simulink model "PartC"  (R2022b)
settings: Solver=ode4  StartTime=0.0  StopTime=1  FixedStep=0.001  RelTol=1e-3
libraries: slpidlib x2
settings Model: PacingRate=0.100000  Creator=Dimuthu  LastModifiedBy=Mushrif
settings DebuggingCC: UnconnectedInputMsg=warning  UnconnectedOutputMsg=warning  UnconnectedLineMsg=warning
settings ModelReferenceCC: EnableRefExpFcnMdlSchedulingChecks=on
settings RTWCC: DLArmComputeVersion=19.05

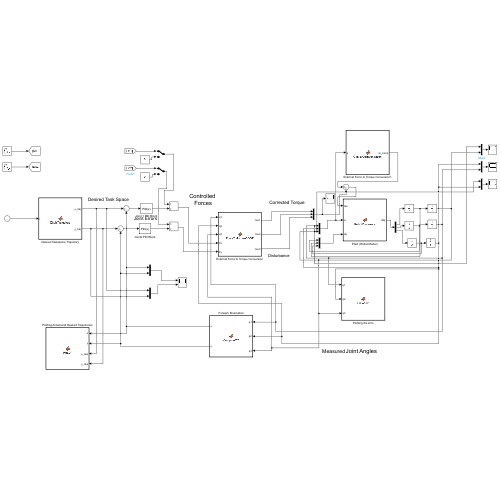
[thumbnail: Simulink's stored preview of the top-level diagram]
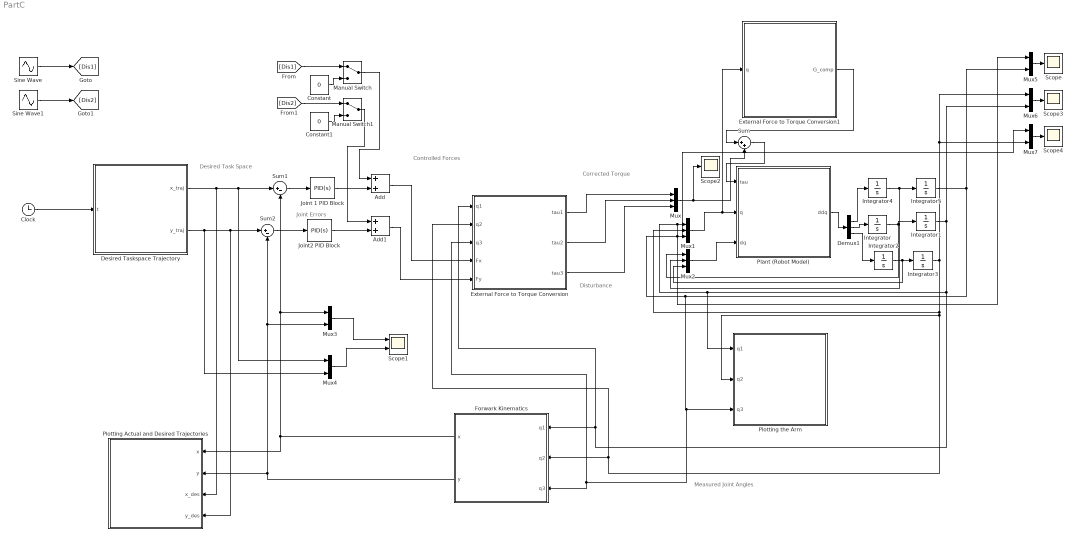
== system PartC ==
  note: Corrected Torque
  note: Disturbance
  note: Measured Joint Angles
  note: Desired Task Space
  note: Controlled
      | Forces
  note: Joint Errors
  Add : Sum
  Add1 : Sum
  Clock : Clock
  Constant : Constant  Value=0
  Constant1 : Constant  Value=0
  Demux1 : Demux  Outputs=3
  Desired Taskspace Trajectory : MATLAB Function  TreatAsAtomicUnit=on
  External Force to Torque Conversion : MATLAB Function  TreatAsAtomicUnit=on
  External Force to Torque Conversion1 : MATLAB Function  TreatAsAtomicUnit=on
  Forwark Kinematics : MATLAB Function  TreatAsAtomicUnit=on
  Integrator{,1..5} (6 alike) : Integrator
  Joint 1 PID Block : slpidlib/PID Controller  Controller=PID  Form=Parallel  TimeDomain=Continuous-time  UseExternalTs=off  SampleTime=-1  IntegratorMethod=Forward Euler  FilterMethod=Forward Euler  ControllerParametersSource=internal  P=100  I=0  UseKiTs=off  D=0  N=100  UseFilter=on  TunerSelectOption=Transfer Function Based (PID Tuner App)  InitialConditionSource=internal  InitialConditionForIntegrator=0  InitialConditionForFilter=0  DifferentiatorICPrevScaledInput=0  ExternalReset=none  TrackingMode=off  Kt=1  LimitOutput=off  SatLimitsSource=internal  UpperSaturationLimit=inf  LowerSaturationLimit=-inf  LinearizeAsGain=on  AntiWindupMode=none  Kb=1  LimitIntegrator=off  UpperIntegratorSaturationLimit=inf  LowerIntegratorSaturationLimit=-inf  POutMin=[]  POutMax=[]  IOutMin=[]  IOutMax=[]  DOutMin=[]  DOutMax=[]  NOutMin=[]  NOutMax=[]  SumOutMin=[]  SumOutMax=[]  SaturationOutMin=[]  SaturationOutMax=[]  PParamMin=[]  PParamMax=[]  IParamMin=[]  IParamMax=[]  DParamMin=[]  DParamMax=[]  NParamMin=[]  NParamMax=[]  KbParamMin=[]  KbParamMax=[]  KtParamMin=[]  KtParamMax=[]  KbOutMin=[]  KbOutMax=[]  KtOutMin=[]  KtOutMax=[]  IntegratorOutMin=[]  IntegratorOutMax=[]  FilterOutMin=[]  FilterOutMax=[]  SumI1OutMin=[]  SumI1OutMax=[]  SumI2OutMin=[]  SumI2OutMax=[]  SumI3OutMin=[]  SumI3OutMax=[]  SumI4OutMin=[]  SumI4OutMax=[]  SumDOutMin=[]  SumDOutMax=[]  DifferentiatorOutMin=[]  DifferentiatorOutMax=[]  FilterDiffOutCoefMin=[]  FilterDiffOutCoefMax=[]  ReciprocalOutMin=[]  ReciprocalOutMax=[]  SumDenOutMin=[]  SumDenOutMax=[]  SumNumOutMin=[]  SumNumOutMax=[]  DivideOutMin=[]  DivideOutMax=[]  UdiffTsProdOutMin=[]  UdiffTsProdOutMax=[]  NTsProdOutMin=[]  NTsProdOutMax=[]  UintegralTsProdOutMin=[]  UintegralTsProdOutMax=[]  UngainTsProdOutMin=[]  UngainTsProdOutMax=[]  ClampingZeroOutDataTypeStr=Inherit: Inherit via back propagation  ClampingZeroOutMin=[]  ClampingZeroOutMax=[]  FilterDenConstantOutDataTypeStr=Inherit: Inherit via back propagation  FilterDenConstantOutMin=[]  FilterDenConstantOutMax=[]  PCopyOutDataTypeStr=Inherit: Inherit via back propagation  PCopyOutMin=[]  PCopyOutMax=[]  NCopyOutDataTypeStr=Inherit: Inherit via back propagation  NCopyOutMin=[]  NCopyOutMax=[]  IntegratorContinuousStateAttributes=''  IntegratorStateMustResolveToSignalObject=off  IntegratorRTWStateStorageClass=Auto  FilterContinuousStateAttributes=''  FilterStateMustResolveToSignalObject=off  FilterRTWStateStorageClass=Auto  ParallelPVariant=InternalParameters  IdealPVariant=Disabled  IVariant=InternalParameters  DVariant=InternalParameters  IntegratorVariant=Continuous  SatVariant=Disabled  AWVariant=Passthrough  PCopyVariant=Disabled  TRVariant=Disabled  FdbkBlocksVariant=Forward  IdealPFdbkVariant=Disabled  SatFdbkVariant=Disabled  DerivativeFilterVariant=ContFilter  NVariant=InternalParameters  NCopyVariant=Disabled  FilterICVariant=InternalICsFilter  IntegratorICVariant=InternalICs  ExternalResetVariant=Disabled  TRSumVariant=Passthrough  SumFdbkVariant=Disabled  SumVariant=Sum_PID  TsampFilterVariant=InternalTs  TsampNgainVariant=Passthrough  TsampIntegralVariant=Passthrough  ExternalSaturationOutDataTypeStr=Inherit: Same as second input
  Joint2 PID Block : slpidlib/PID Controller  Controller=PID  Form=Parallel  TimeDomain=Continuous-time  UseExternalTs=off  SampleTime=-1  IntegratorMethod=Forward Euler  FilterMethod=Forward Euler  ControllerParametersSource=internal  P=10  I=0  UseKiTs=off  D=0  N=100  UseFilter=on  TunerSelectOption=Transfer Function Based (PID Tuner App)  InitialConditionSource=internal  InitialConditionForIntegrator=0  InitialConditionForFilter=0  DifferentiatorICPrevScaledInput=0  ExternalReset=none  TrackingMode=off  Kt=1  LimitOutput=off  SatLimitsSource=internal  UpperSaturationLimit=inf  LowerSaturationLimit=-inf  LinearizeAsGain=on  AntiWindupMode=none  Kb=1  LimitIntegrator=off  UpperIntegratorSaturationLimit=inf  LowerIntegratorSaturationLimit=-inf  POutMin=[]  POutMax=[]  IOutMin=[]  IOutMax=[]  DOutMin=[]  DOutMax=[]  NOutMin=[]  NOutMax=[]  SumOutMin=[]  SumOutMax=[]  SaturationOutMin=[]  SaturationOutMax=[]  PParamMin=[]  PParamMax=[]  IParamMin=[]  IParamMax=[]  DParamMin=[]  DParamMax=[]  NParamMin=[]  NParamMax=[]  KbParamMin=[]  KbParamMax=[]  KtParamMin=[]  KtParamMax=[]  KbOutMin=[]  KbOutMax=[]  KtOutMin=[]  KtOutMax=[]  IntegratorOutMin=[]  IntegratorOutMax=[]  FilterOutMin=[]  FilterOutMax=[]  SumI1OutMin=[]  SumI1OutMax=[]  SumI2OutMin=[]  SumI2OutMax=[]  SumI3OutMin=[]  SumI3OutMax=[]  SumI4OutMin=[]  SumI4OutMax=[]  SumDOutMin=[]  SumDOutMax=[]  DifferentiatorOutMin=[]  DifferentiatorOutMax=[]  FilterDiffOutCoefMin=[]  FilterDiffOutCoefMax=[]  ReciprocalOutMin=[]  ReciprocalOutMax=[]  SumDenOutMin=[]  SumDenOutMax=[]  SumNumOutMin=[]  SumNumOutMax=[]  DivideOutMin=[]  DivideOutMax=[]  UdiffTsProdOutMin=[]  UdiffTsProdOutMax=[]  NTsProdOutMin=[]  NTsProdOutMax=[]  UintegralTsProdOutMin=[]  UintegralTsProdOutMax=[]  UngainTsProdOutMin=[]  UngainTsProdOutMax=[]  ClampingZeroOutDataTypeStr=Inherit: Inherit via back propagation  ClampingZeroOutMin=[]  ClampingZeroOutMax=[]  FilterDenConstantOutDataTypeStr=Inherit: Inherit via back propagation  FilterDenConstantOutMin=[]  FilterDenConstantOutMax=[]  PCopyOutDataTypeStr=Inherit: Inherit via back propagation  PCopyOutMin=[]  PCopyOutMax=[]  NCopyOutDataTypeStr=Inherit: Inherit via back propagation  NCopyOutMin=[]  NCopyOutMax=[]  IntegratorContinuousStateAttributes=''  IntegratorStateMustResolveToSignalObject=off  IntegratorRTWStateStorageClass=Auto  FilterContinuousStateAttributes=''  FilterStateMustResolveToSignalObject=off  FilterRTWStateStorageClass=Auto  ParallelPVariant=InternalParameters  IdealPVariant=Disabled  IVariant=InternalParameters  DVariant=InternalParameters  IntegratorVariant=Continuous  SatVariant=Disabled  AWVariant=Passthrough  PCopyVariant=Disabled  TRVariant=Disabled  FdbkBlocksVariant=Forward  IdealPFdbkVariant=Disabled  SatFdbkVariant=Disabled  DerivativeFilterVariant=ContFilter  NVariant=InternalParameters  NCopyVariant=Disabled  FilterICVariant=InternalICsFilter  IntegratorICVariant=InternalICs  ExternalResetVariant=Disabled  TRSumVariant=Passthrough  SumFdbkVariant=Disabled  SumVariant=Sum_PID  TsampFilterVariant=InternalTs  TsampNgainVariant=Passthrough  TsampIntegralVariant=Passthrough  ExternalSaturationOutDataTypeStr=Inherit: Same as second input
  Manual Switch : ManualSwitch
  Manual Switch1 : ManualSwitch
  Mux : Mux  Inputs=3
  Mux1 : Mux  Inputs=3
  Mux2 : Mux  Inputs=3
  Mux{3..7} (5 alike) : Mux  Inputs=2
  Plant (Robot Model) : MATLAB Function  TreatAsAtomicUnit=on
  Plotting Actual and Desired Trajectories : MATLAB Function  TreatAsAtomicUnit=on
  Plotting the Arm : MATLAB Function  TreatAsAtomicUnit=on
  Scope{,2..4} (4 alike) : Scope
  Scope1 : Scope  NumInputPorts=2
  Sine Wave : Sin  Amplitude=0.1  SampleTime=0
  Sine Wave1 : Sin  Amplitude=0.05  SampleTime=0
  Sum : Sum  Inputs=|++
  Sum1 : Sum  Inputs=|+-
  Sum2 : Sum  Inputs=|+-
  wires:
  Desired Taskspace Trajectory/1(x_traj) -> Plotting Actual and Desired Trajectories/3(x_des), Mux4/1, Sum1/1
  Desired Taskspace Trajectory/2(y_traj) -> Mux4/2, Plotting Actual and Desired Trajectories/4(y_des), Sum2/1
  Forwark Kinematics/1(x) -> Mux3/1, Sum1/2, Plotting Actual and Desired Trajectories/1(x)
  Forwark Kinematics/2(y) -> Plotting Actual and Desired Trajectories/2(y), Mux3/2, Sum2/2
  Sum2/1 -> Joint2 PID Block/1
  Sum1/1 -> Joint 1 PID Block/1
  External Force to Torque Conversion/1(tau1) -> Mux/1
  Integrator/1 -> Integrator1/1, Mux2/1
  Demux1/2 -> Integrator/1
  Demux1/3 -> Integrator2/1
  Integrator2/1 -> Mux2/3, Integrator3/1
  Mux1/1 -> External Force to Torque Conversion1/1(q), Plant (Robot Model)/2(q)
  Mux2/1 -> Plant (Robot Model)/3(dq)
  Integrator1/1 -> Mux6/2, Mux5/1, Mux1/1, Plotting the Arm/1(q1), External Force to Torque Conversion/1(q1), Forwark Kinematics/1(q1)
  Integrator3/1 -> Mux6/1, Mux7/2, Mux1/2, Plotting the Arm/2(q2), External Force to Torque Conversion/2(q2), Forwark Kinematics/2(q2)
  Plant (Robot Model)/1(ddq) -> Demux1/1
  Mux3/1 -> Scope1/1
  Mux4/1 -> Scope1/2
  Mux/1 -> Sum/2, Scope2/1
  External Force to Torque Conversion/2(tau2) -> Mux/2
  Demux1/1 -> Integrator4/1
  Integrator4/1 -> Mux2/2, Integrator5/1
  Integrator5/1 -> Mux5/2, Forwark Kinematics/3(q3), External Force to Torque Conversion/3(q3), Plotting the Arm/3(q3), Mux7/1, Mux1/3
  External Force to Torque Conversion/3(tau3) -> Mux/3
  Clock/1 -> Desired Taskspace Trajectory/1(t)
  External Force to Torque Conversion1/1(G_comp) -> Sum/1
  Sum/1 -> Plant (Robot Model)/1(tau)
  Mux5/1 -> Scope/1
  Mux6/1 -> Scope3/1
  Mux7/1 -> Scope4/1
  Joint2 PID Block/1 -> Add1/2
  Joint 1 PID Block/1 -> Add/2
  Add/1 -> External Force to Torque Conversion/4(Fx)
  Add1/1 -> External Force to Torque Conversion/5(Fy)
  Sine Wave/1 -> [Dis1]
  Sine Wave1/1 -> [Dis2]
  Manual Switch1/1 -> Add1/1
  Manual Switch/1 -> Add/1
  [Dis1] -> Manual Switch/1
  [Dis2] -> Manual Switch1/1
  Constant1/1 -> Manual Switch1/2
  Constant/1 -> Manual Switch/2

== matlab function PartC/Forwark Kinematics ==
  settings: updateMethod=DISCRETE
  data: q1 input double size=1; q2 input double size=1; x output; y output; q3 input
function [x, y] = ComputeXY(q1, q2, q3)
%#codegen

% Define link lengths (can be parameters later)
l1 = 0.5; l2 = 0.4; l3 = 0.3;

% Compute forward kinematics
x = l1 * cos(q1) + l2 * cos(q1 + q2)+ l3 * cos(q1 + q2 + q3);
y = l1 * sin(q1) + l2 * sin(q1 + q2)+ l3 * sin(q1 + q2 + q3);
end

== matlab function PartC/Desired Taskspace Trajectory ==
  settings: updateMethod=DISCRETE
  data: x_traj output; y_traj output; t input
function [x_traj, y_traj] = CircleTrajectory(t)
T = 1;             % total time
%dt = 0.05;          % time step
%t = 0:dt:T;
%N = length(t);

% Robot planar workspace: max reach = 0.5 + 0.4 + 0.3 = 1.2 m
% Set a reachable elliptical trajectory in the XY plane
cx = 0.9; cy = 0.3;           % center of ellipse
rx = 0.3; ry = 0.2;           % radii (x and y)
%rx = 0.8; ry = 0.4; 

% 2D elliptical arc in XY plane
x_traj = cx + rx * cos(2*pi*t/T);
y_traj = cy + ry * sin(2*pi*t/T);
end

== matlab function PartC/External Force to Torque Conversion ==
  settings: updateMethod=DISCRETE
  data: q1 input double size=[1,1]; q2 input double size=[1,1]; q3 input size=[1,1]; tau1 output size=[1,1]; tau2 output size=[1,1]; Fx input size=[1,1]; Fy input size=[1,1]; tau3 output size=[1,1]
function [tau1, tau2, tau3] = ForceToTorque3DOF(q1, q2, q3, Fx, Fy)
% Converts end-effector force to joint torques for a 3-DOF planar robot.
% Safer version without damping or dq input.

% Link lengths
l1 = 0.5; l2 = 0.4; l3 = 0.3;

% === Wrap angles to avoid large angle buildup ===
q1 = wrapToPi(q1);
q2 = wrapToPi(q2);
q3 = wrapToPi(q3);

% === Force saturation to avoid instability ===
Fmax = 100;  % Tune as needed
Fx = max(min(Fx, Fmax), -Fmax);
Fy = max(min(Fy, Fmax), -Fmax);

F_ee = [Fx; Fy];  % Cartesian force

% === Trigonometric precomputations ===
s1 = sin(q1); c1 = cos(q1);
s12 = sin(q1 + q2); c12 = cos(q1 + q2);
s123 = sin(q1 + q2 + q3); c123 = cos(q1 + q2 + q3);

% === Jacobian (2x3) ===
J11 = -l1*s1 - l2*s12 - l3*s123;
J12 =       -l2*s12 - l3*s123;
J13 =                 -l3*s123;

J21 =  l1*c1 + l2*c12 + l3*c123;
J22 =         l2*c12 + l3*c123;
J23 =                  l3*c123;

J = [J11 J12 J13;
     J21 J22 J23];

% === Check Jacobian and force validity ===
if any(~isfinite(J(:))) || any(~isfinite(F_ee))
    tau_vec = [0; 0; 0];  % Failsafe zero torque
else
    tau_vec = J' * F_ee;
end

% === Output joint torques ===
tau1 = tau_vec(1);
tau2 = tau_vec(2);
tau3 = tau_vec(3);
end

== matlab function PartC/Plant (Robot Model) ==
  data: tau input double size=[3,1]; q input double size=[3,1]; dq input size=[3,1]; ddq output size=[3,1]
function ddq = RobotDynamics(tau, q, dq)
% 3-DOF Planar Robot Dynamics - ROBUST VERSION
% Inputs:
%   tau - joint torques [3x1]
%   q   - joint positions [3x1]
%   dq  - joint velocities [3x1]
% Output:
%   ddq - joint accelerations [3x1]

% --- Ensure inputs are column vectors ---
q = q(:);
dq = dq(:);
tau = tau(:);

% --- Robot parameters (MUST MATCH ALL OTHER BLOCKS) ---
m1 = 1; m2 = 1; m3 = 1;
l1 = 0.5; l2 = 0.4; l3 = 0.3;
%l1 = 0.1; l2 = 0.1;l3 = 0.1;
g = 9.81;

% === Inertia Matrix M(q) ===
M11 = m1*l1^2 + m2*(l1^2 + l2^2 + 2*l1*l2*cos(q(2))) + ...
      m3*(l1^2 + l2^2 + l3^2 + 2*l1*l2*cos(q(2)) + 2*l1*l3*cos(q(2)+q(3)) + 2*l2*l3*cos(q(3)));
M12 = m2*(l2^2 + l1*l2*cos(q(2))) + ...
      m3*(l2^2 + l3^2 + l1*l2*cos(q(2)) + l1*l3*cos(q(2)+q(3)) + l2*l3*cos(q(3)));
M13 = m3*(l3^2 + l1*l3*cos(q(2)+q(3)) + l2*l3*cos(q(3)));
M22 = m2*l2^2 + m3*(l2^2 + l3^2 + 2*l2*l3*cos(q(3)));
M23 = m3*(l3^2 + l2*l3*cos(q(3)));
M33 = m3*l3^2;
M = [M11 M12 M13;
     M12 M22 M23;
     M13 M23 M33];

% === Coriolis and Centripetal Matrix C(q,dq) ===
c1 = -m2*l1*l2*sin(q(2))*(2*dq(1)*dq(2) + dq(2)^2) ...
     - m3*(l1*l2*sin(q(2))*(2*dq(1)*dq(2) + dq(2)^2) ...
     + l1*l3*sin(q(2)+q(3))*(2*dq(1)*(dq(2)+dq(3)) + (dq(2)+dq(3))^2) ...
     + l2*l3*sin(q(3))*(2*dq(2)*dq(3) + dq(3)^2));
c2 = m2*l1*l2*sin(q(2))*dq(1)^2 + ...
     m3*(l1*l2*sin(q(2))*dq(1)^2 + ...
     l1*l3*sin(q(2)+q(3))*dq(1)^2 + ...
     l2*l3*sin(q(3))*(2*dq(2)*dq(3) + dq(3)^2));
c3 = m3*(l1*l3*sin(q(2)+q(3))*dq(1)^2 + ...
         l2*l3*sin(q(3))*dq(2)^2);
C = [c1; c2; c3];

% === Gravity Vector G(q) ===
G1 = g*(m1*l1*cos(q(1)) + m2*(l1*cos(q(1)) + l2*cos(q(1)+q(2))) + ...
        m3*(l1*cos(q(1)) + l2*cos(q(1)+q(2)) + l3*cos(q(1)+q(2)+q(3))));
G2 = g*(m2*l2*cos(q(1)+q(2)) + m3*(l2*cos(q(1)+q(2)) + l3*cos(q(1)+q(2)+q(3))));
G3 = g*(m3*l3*cos(q(1)+q(2)+q(3)));
G = [G1; G2; G3];

% =================================================================
% === MODIFICATIONS FOR STABILITY =================================
% =================================================================

% --- MODIFICATION 1: Add Joint Damping ---
% This adds physical realism (friction) and helps stabilize the system.
% Tune these values if needed. Higher values = more "syrupy" motion.
D = diag([0.5, 0.5, 0.5]);
DampingTorque = D * dq;

% --- MODIFICATION 2: Regularize the Inertia Matrix ---
% This is the direct fix for the singularity crash.
% It adds a tiny value to the diagonal of M, guaranteeing it is
% always invertible and preventing the ddq calculation from failing.
epsilon = 1e-6; % A small number
M_reg = M + epsilon * eye(size(M));

% --- Calculate the net torque on the system ---
% We subtract Coriolis, Gravity, and the new Damping torques.
residual_torque = tau - C - G - DampingTorque;

% --- Final Robust Calculation of ddq ---
% Use the regularized matrix M_reg to avoid crashes.
ddq = M_reg \ residual_torque;

% --- Failsafe Guard ---
% If for any reason ddq is still not finite, output zeros to
% prevent the entire simulation from stopping.
if any(~isfinite(ddq))
    ddq = zeros(3,1);
end

end

== matlab function PartC/Plotting the Arm ==
  settings: updateMethod=DISCRETE
  data: q1 input double size=1; q2 input double size=1; q3 input
function DrawArm(q1, q2, q3)
% DrawArm - Plots a 3-DOF planar robot arm in 2D
% Inputs: q1, q2, q3 - joint angles (in radians)

% Link lengths
l1 = 0.5; l2 = 0.4; l3 = 0.3;

% Forward kinematics
x1 = l1 * cos(q1);
y1 = l1 * sin(q1);

x2 = x1 + l2 * cos(q1 + q2);
y2 = y1 + l2 * sin(q1 + q2);

x3 = x2 + l3 * cos(q1 + q2 + q3);
y3 = y2 + l3 * sin(q1 + q2 + q3);

% Persistent graphics handles
persistent h1 h2 h3 base initialized
if isempty(initialized)
    figure(1); clf;
    axis equal; axis([-3.5 3.5 -3.5 3.5]);
    grid on; hold on;
    base = plot(0, 0, 'ko', 'MarkerSize', 6, 'MarkerFaceColor', 'k');
    h1 = plot([0, x1], [0, y1], 'r-', 'LineWidth', 5);       % Link 1
    h2 = plot([x1, x2], [y1, y2], 'g-', 'LineWidth', 5);     % Link 2
    h3 = plot([x2, x3], [y2, y3], 'b-', 'LineWidth', 5);     % Link 3
    initialized = true;
else
    set(h1, 'XData', [0, x1], 'YData', [0, y1]);
    set(h2, 'XData', [x1, x2], 'YData', [y1, y2]);
    set(h3, 'XData', [x2, x3], 'YData', [y2, y3]);
end

drawnow;
end

== matlab function PartC/Plotting Actual and Desired Trajectories ==
  settings: updateMethod=DISCRETE
  data: x input double size=1; y input double size=1; x_des input; y_des input
function PlotXY(x, y, x_des, y_des)
%#codegen

persistent h_actual h_des trail_x trail_y trail_xd trail_yd idx initialized
if isempty(initialized)
    figure(2); clf;
    axis equal; axis([0 2 -1.2 1.2]);
    grid on; hold on;

    h_actual = plot(nan, nan, 'b-', 'LineWidth', 2); % Actual path
    h_des    = plot(nan, nan, 'r--', 'LineWidth', 2); % Desired path

    N = 10000;
    trail_x = nan(N,1);
    trail_y = nan(N,1);
    trail_xd = nan(N,1);
    trail_yd = nan(N,1);
    idx = 1;

    initialized = true;
end

if idx <= length(trail_x)
    trail_x(idx)  = x;
    trail_y(idx)  = y;
    trail_xd(idx) = x_des;
    trail_yd(idx) = y_des;

    set(h_actual, 'XData', trail_x,  'YData', trail_y);
    set(h_des,    'XData', trail_xd, 'YData', trail_yd);

    idx = idx + 1;
end

drawnow limitrate;
end

== matlab function PartC/External Force to Torque Conversion1 ==
  settings: updateMethod=DISCRETE
  data: q input double size=[1,3]; G_comp output size=[3]
function G_comp = GravityCompensation(q)
% Calculates the gravity compensation torque vector G(q).
% This block computes the torques required to hold the robot's
% position against gravity.
%
% Input:
%   q      - A 3x1 vector of current joint angles [q1; q2; q3].
% Output:
%   G_comp - A 3x1 vector of gravity torques [G1; G2; G3].

% --- Ensure input is a column vector to prevent dimension errors ---
% This is a safety measure for Simulink.
q = q(:);

% --- Robot Parameters ---
% IMPORTANT: These parameters MUST exactly match the ones in your
% RobotDynamics.m file for the compensation to be effective.
m1 = 1; m2 = 1; m3 = 1;
l1 = 0.5; l2 = 0.4; l3 = 0.3;
g = 9.81;

% --- Gravity Vector G(q) Calculation ---
% This is the exact same logic as in your RobotDynamics file.
% It calculates the torque on each joint due to gravity.
G1 = g * (m1*l1*cos(q(1)) + m2*(l1*cos(q(1)) + l2*cos(q(1)+q(2))) + ...
         m3*(l1*cos(q(1)) + l2*cos(q(1)+q(2)) + l3*cos(q(1)+q(2)+q(3))));

G2 = g * (m2*l2*cos(q(1)+q(2)) + m3*(l2*cos(q(1)+q(2)) + l3*cos(q(1)+q(2)+q(3))));

G3 = g * (m3*l3*cos(q(1)+q(2)+q(3)));

% --- Define the output vector ---
% This vector will be added to the controller's output torque.
G_comp = [G1; G2; G3];

end
